simulink model "ThrottleValveController"  (R2024b)
settings: Solver=VariableStepAuto  StartTime=0.0  StopTime=10.0  RelTol=1e-3
libraries: slpidlib x1
settings Model: DataDictionary=SysMLArchModel_DD.sldd  Creator=ykamatan  LastModifiedBy=hnakano

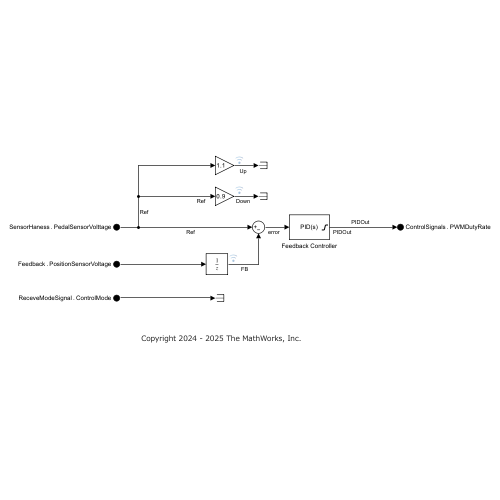
[thumbnail: Simulink's stored preview of the top-level diagram]
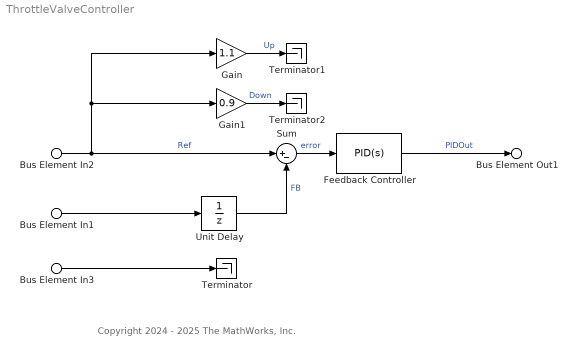
== system ThrottleValveController ==
  note: Copyright 2024 - 2025 The MathWorks, Inc.
  Bus Element In1 : Inport  PortName=Feedback  Element=PositionSensorVoltage
  Bus Element In2 : Inport  Port=2  PortName=SensorHaness  Element=PedalSensorVolttage
  Bus Element In3 : Inport  Port=3  PortName=ReceveModeSignal  Element=ControlMode
  Feedback Controller : slpidlib/PID Controller  Controller=PID  Form=Ideal  TimeDomain=Continuous-time  UseExternalTs=off  SampleTime=-1  IntegratorMethod=Forward Euler  FilterMethod=Forward Euler  ControllerParametersSource=internal  P=0.035  I=0.7  UseKiTs=off  D=0.028  UseExternalDerivativeSource=off  N=100  UseFilter=on  TunerSelectOption=Transfer Function Based (PID Tuner App)  InitialConditionSource=internal  InitialConditionForIntegrator=0  InitialConditionForFilter=0  DifferentiatorICPrevScaledInput=0  ExternalReset=none  TrackingMode=off  Kt=1  LimitOutput=on  SatLimitsSource=internal  UpperSaturationLimit=0.90  LowerSaturationLimit=0  LinearizeAsGain=off  AntiWindupMode=back-calculation  Kb=1  LimitIntegrator=off  UpperIntegratorSaturationLimit=inf  LowerIntegratorSaturationLimit=-inf  POutMin=[]  POutMax=[]  IOutMin=[]  IOutMax=[]  DOutMin=[]  DOutMax=[]  NOutMin=[]  NOutMax=[]  SumOutMin=[]  SumOutMax=[]  SaturationOutMin=[]  SaturationOutMax=[]  PParamMin=[]  PParamMax=[]  IParamMin=[]  IParamMax=[]  DParamMin=[]  DParamMax=[]  NParamMin=[]  NParamMax=[]  KbParamMin=[]  KbParamMax=[]  KtParamMin=[]  KtParamMax=[]  KbOutMin=[]  KbOutMax=[]  KtOutMin=[]  KtOutMax=[]  IntegratorOutMin=[]  IntegratorOutMax=[]  FilterOutMin=[]  FilterOutMax=[]  SumI1OutMin=[]  SumI1OutMax=[]  SumI2OutMin=[]  SumI2OutMax=[]  SumI3OutMin=[]  SumI3OutMax=[]  SumI4OutMin=[]  SumI4OutMax=[]  SumDOutMin=[]  SumDOutMax=[]  DifferentiatorOutMin=[]  DifferentiatorOutMax=[]  FilterDiffOutCoefMin=[]  FilterDiffOutCoefMax=[]  ReciprocalOutMin=[]  ReciprocalOutMax=[]  SumDenOutMin=[]  SumDenOutMax=[]  SumNumOutMin=[]  SumNumOutMax=[]  DivideOutMin=[]  DivideOutMax=[]  UdiffTsProdOutMin=[]  UdiffTsProdOutMax=[]  NTsProdOutMin=[]  NTsProdOutMax=[]  UintegralTsProdOutMin=[]  UintegralTsProdOutMax=[]  UngainTsProdOutMin=[]  UngainTsProdOutMax=[]  ClampingZeroOutDataTypeStr=Inherit: Inherit via back propagation  ClampingZeroOutMin=[]  ClampingZeroOutMax=[]  FilterDenConstantOutDataTypeStr=Inherit: Inherit via back propagation  FilterDenConstantOutMin=[]  FilterDenConstantOutMax=[]  PCopyOutDataTypeStr=Inherit: Inherit via back propagation  PCopyOutMin=[]  PCopyOutMax=[]  NCopyOutDataTypeStr=Inherit: Inherit via back propagation  NCopyOutMin=[]  NCopyOutMax=[]  IntegratorContinuousStateAttributes=''  IntegratorStateMustResolveToSignalObject=off  IntegratorRTWStateStorageClass=Auto  FilterContinuousStateAttributes=''  FilterStateMustResolveToSignalObject=off  FilterRTWStateStorageClass=Auto  ParallelPVariant=Passthrough  IdealPVariant=InternalParameters  IVariant=InternalParameters  DVariant=InternalParameters  IntegratorVariant=Continuous  SatVariant=Enabled  AWVariant=BackCalculation  PCopyVariant=Disabled  TRVariant=Disabled  FdbkBlocksVariant=Forward  IdealPFdbkVariant=Disabled  SatFdbkVariant=Disabled  DerivativeFilterVariant=ContFilter  NVariant=InternalParameters  NCopyVariant=Disabled  FilterICVariant=InternalICsFilter  IntegratorICVariant=InternalICs  ExternalResetVariant=Disabled  TRSumVariant=Passthrough  SumFdbkVariant=Disabled  SumVariant=Sum_PID  TsampFilterVariant=InternalTs  TsampNgainVariant=Passthrough  TsampIntegralVariant=Disabled_SignalSpec  ExternalSaturationOutDataTypeStr=Inherit: Same as second input  DerivativeSourceVariant=ErrorSignal  PreIntVariant=InternalPreInt
  Gain : Gain  Gain=1.1
  Gain1 : Gain  Gain=0.9
  Sum : Sum  Inputs=|+-
  Terminator : Terminator
  Terminator1 : Terminator
  Terminator2 : Terminator
  Unit Delay : UnitDelay  SampleTime=1/10000  HasFrameUpgradeWarning=on
  Bus Element Out1 : Outport  PortName=ControlSignals  Element=PWMDutyRate
  wires:
  Unit Delay/1 -> Sum/2  "FB"
  Sum/1 -> Feedback Controller/1  "error"
  Gain1/1 -> Terminator2/1  "Down"
  Feedback Controller/1 -> Bus Element Out1/1  "PIDOut"
  Bus Element In2/1 -> Gain1/1, Gain/1, Sum/1  "Ref"
  Bus Element In3/1 -> Terminator/1
  Gain/1 -> Terminator1/1  "Up"
  Bus Element In1/1 -> Unit Delay/1
